simulink model "AeropendulumNonLinearModel"  (R2025b)
settings: Solver=VariableStepAuto  StartTime=0.0  StopTime=600  RelTol=1e-3
values from neighbouring files (symbols this model uses):
  b = 0.05    [datos_procesados.mat]    (also in linearization.m; modelId.m; pid_design.m; tratamiento_datos.m)
  J = 0.000448229    [datos_procesados.mat]    (also in linearization.m; modelId.m; pid_design.m; tratamiento_datos.m)
  mgl = 0.02672244    [datos_procesados.mat]    (also in linearization.m; modelId.m; pid_design.m; tratamiento_datos.m)
  T_lut = [0 0 0 0 0 4.09916934892e-05 0.000327925445548 0.000573839821716 0.000983578806617 0.00147495160542 0.00266004837703 0.00331179149163 ... (51 elements, 51x1)]    [datos_procesados.mat]    (also in tratamiento_datos.m = [Tl; T_ext]; voltTorque.m = T_lut_ext; voltTorque_Descendiente.m = T_lut_ext; voltTorque_v2.m = q(2)*max(V_lut - q(3), 0).^q(4))
  V_lut = [0 0.1 0.2 0.3 0.4 0.5 0.6 0.7 0.8 0.9 1 1.1 ... (51 elements, 51x1)]    [datos_procesados.mat]    (also in tratamiento_datos.m = [Vl; V_ext]; voltTorque.m = V_lut_ext; voltTorque_Descendiente.m = V_lut_ext; voltTorque_v2.m = (0:0.05:5)')
libraries: simulink x2
settings Model: Creator=Anon  LastModifiedBy=Anon

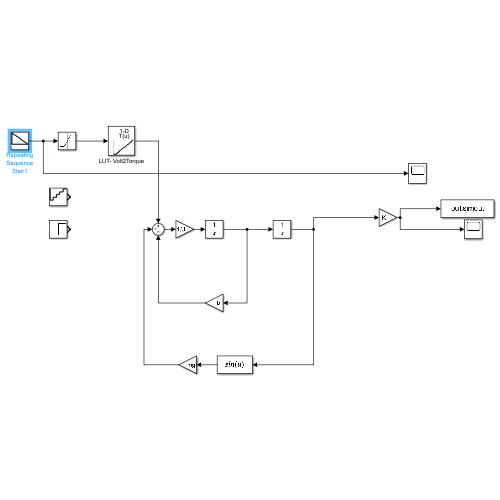
[thumbnail: Simulink's stored preview of the top-level diagram]
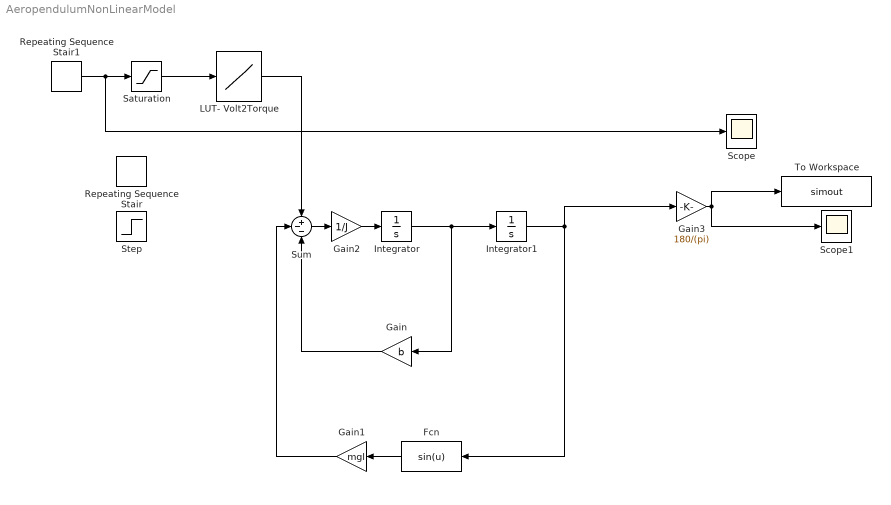
== system AeropendulumNonLinearModel ==
  Fcn : Fcn  Expr=sin(u)
  Gain : Gain  Gain=b
  Gain1 : Gain  Gain=mgl
  Gain2 : Gain  Gain=1/J
  Gain3 : Gain  Gain=180/(pi)
  Integrator : Integrator
  Integrator1 : Integrator  InitialCondition=pi/2
  LUT- Volt2Torque : Lookup_n-D  NumberOfTableDimensions=1  BreakpointsForDimension1=V_lut  BeginIndexSearchUsingPreviousIndexResult=on  Table=T_lut  InternalRulePriority=Speed  RndMeth=Simplest
  Repeating Sequence Stair : simulink/Sources/Repeating Sequence Stair  OutValues=[0.005 0.01 0.015 0.02 0.025].'  tsamp=20  OutMin=[]  OutMax=[]  OutDataTypeStr=double  OutputDataTypeScalingMode=double  OutDataType=fixdt(0,8)  ConRadixGroup=Best Precision: Vector-wise  OutScaling=2^-12
  Repeating Sequence Stair1 : simulink/Sources/Repeating Sequence Stair  OutValues=voltageProfileDesc  tsamp=sampleTime  OutMin=[]  OutMax=[]  OutDataTypeStr=double  OutputDataTypeScalingMode=double  OutDataType=fixdt(0,8)  ConRadixGroup=Best Precision: Vector-wise  OutScaling=2^-12
  Saturation : Saturate  UpperLimit=5  LowerLimit=0
  Scope : Scope
      settings: ActiveDisplayYMinimum=-0.5874999999999998  ActiveDisplayYMaximum=5.2875  DataLoggingVariableName=mod_pwm
  Scope1 : Scope
      settings: ActiveDisplayYMinimum=-11.250130278113307  ActiveDisplayYMaximum=101.25001447534592  DataLoggingVariableName=mod_angle
  Step : Step  After=0.005  SampleTime=0
  Sum : Sum  Inputs=+--
  To Workspace : ToWorkspace  VariableName=simout  SaveFormat=Timeseries  SampleTime=-1
  wires:
  Integrator/1 -> Gain/1, Integrator1/1
  Gain/1 -> Sum/3
  Integrator1/1 -> Fcn/1, Gain3/1
  Fcn/1 -> Gain1/1
  Gain1/1 -> Sum/2
  LUT- Volt2Torque/1 -> Sum/1
  Gain3/1 -> To Workspace/1, Scope1/1
  Sum/1 -> Gain2/1
  Gain2/1 -> Integrator/1
  Repeating Sequence Stair1/1 -> Scope/1, Saturation/1
  Saturation/1 -> LUT- Volt2Torque/1
